simulink model "npc_diag"  (R2023b)
settings: Solver=FixedStepDiscrete  StartTime=0  StopTime=4  FixedStep=1e-06  RelTol=1e-3
libraries: spsThreePhaseSeriesRLCBranchLib x3, spsDCVoltageSourceLib x2, spsVoltageMeasurementLib x2, spsGroundLib x1, spsThreeLevelBridgeLib x1, spsPWMGenerator3LevelLib x1, spsThreePhaseVIMeasurementLib x1, spspowerguiLib x1
settings Model: Creator=ASUS  LastModifiedBy=ASUS
settings DataIOCC: SaveOutput=off  SaveTime=off

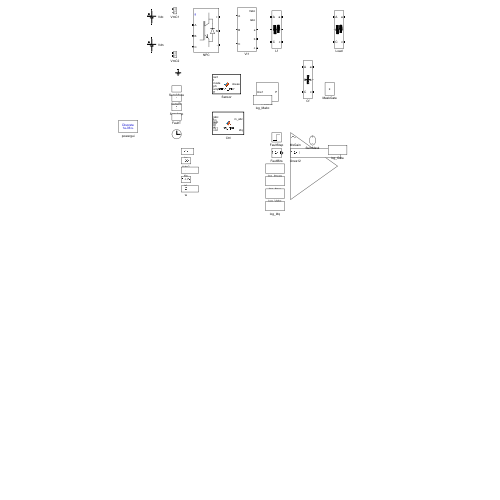
[thumbnail: Simulink's stored preview of the top-level diagram]
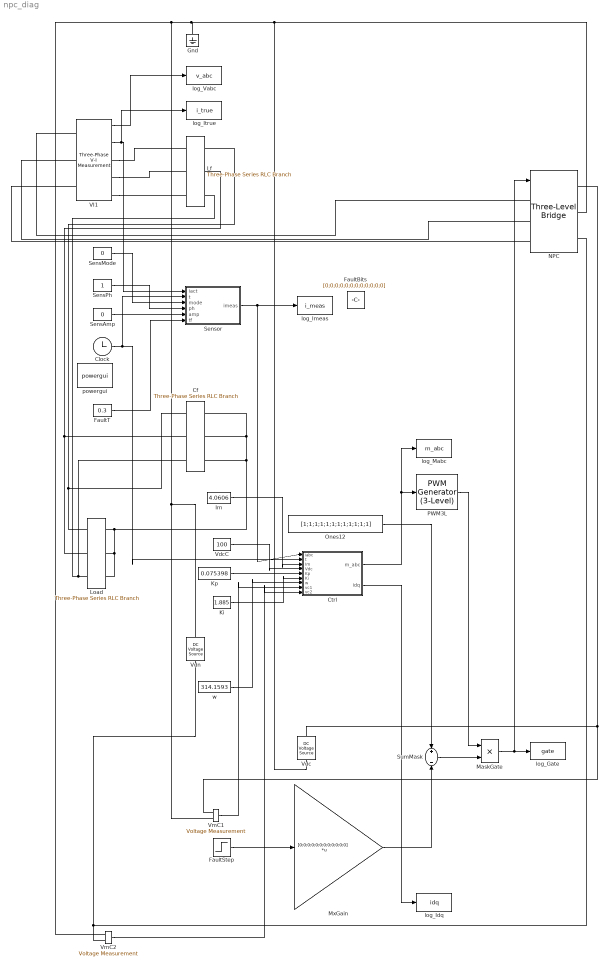
== system npc_diag ==
  Cf : spsThreePhaseSeriesRLCBranchLib/Three-Phase Series RLC Branch  LConnTagsString=A|B|C  RConnTagsString=A|B|C  BranchType=C  Resistance=1  Inductance=1e-3  Capacitance=5e-05  Measurements=None
  Clock : Clock
  Ctrl : MATLAB Function  TreatAsAtomicUnit=on
  FaultBits : Constant  Value=[0;0;0;0;0;0;0;0;0;0;0;0]
  FaultStep : Step  Time=0.3  SampleTime=0
  FaultT : Constant  Value=0.3
  Gnd : spsGroundLib/Ground  LConnTagsString=a
  Im : Constant  Value=4.0606
  Ki : Constant  Value=1.885
  Kp : Constant  Value=0.075398
  Lf : spsThreePhaseSeriesRLCBranchLib/Three-Phase Series RLC Branch  LConnTagsString=A|B|C  RConnTagsString=A|B|C  BranchType=RL  Resistance=0.05  Inductance=0.002  Capacitance=1e-6  Measurements=None
  Load : spsThreePhaseSeriesRLCBranchLib/Three-Phase Series RLC Branch  LConnTagsString=A|B|C  RConnTagsString=A|B|C  BranchType=RL  Resistance=10  Inductance=0  Capacitance=1e-6  Measurements=None
  MaskGate : Product
  MxGain : Gain  Gain=[0;0;0;0;0;0;0;0;0;0;0;0]  Multiplication=Matrix(K*u)
  NPC : spsThreeLevelBridgeLib/Three-Level Bridge  Arms=3  SnubberResistance=100000  SbubberCapacitance=inf  Device=IGBT / Diodes  Ron=0.001  ForwardVoltages=[0 0]  Measurements=None
  Ones12 : Constant  Value=[1;1;1;1;1;1;1;1;1;1;1;1]
  PWM3L : spsPWMGenerator3LevelLib/PWM Generator (3-Level)  ModulatorType=Three-phase bridge (12 pulses)  ModulatorMode=Unsynchronized  nF=200  Fc=10000  ModulatingSignals=off  m=0.8  Freq=50  Phase=0  Ts=0
  SensAmp : Constant  Value=0
  SensMode : Constant  Value=0
  SensPh : Constant
  Sensor : MATLAB Function  TreatAsAtomicUnit=on
  SumMask : Sum  Inputs=+-
  VI1 : spsThreePhaseVIMeasurementLib/Three-Phase V-I Measurement  VoltageMeasurement=phase-to-ground  SetLabelV=off  LabelV=Vabc  Vpu=off  VpuLL=off  CurrentMeasurement=yes  SetLabelI=off  LabelI=Iabc  Ipu=off  Pbase=100e6  Vbase=500e3  OutputType=Complex  PhasorSimulation=off  PSBequivalent=0
  Vdc : spsDCVoltageSourceLib/DC Voltage Source  Amplitude=50  Measurements=None
  VdcC : Constant  Value=100
  Vdn : spsDCVoltageSourceLib/DC Voltage Source  Amplitude=50  Measurements=None
  VmC1 : spsVoltageMeasurementLib/Voltage Measurement  PhasorSimulation=off  OutputType=Complex  PSBequivalent=0
  VmC2 : spsVoltageMeasurementLib/Voltage Measurement  PhasorSimulation=off  OutputType=Complex  PSBequivalent=0
  log_Gate : ToWorkspace  VariableName=gate  SaveFormat=Timeseries  SampleTime=5e-05
  log_Idq : ToWorkspace  VariableName=idq  SaveFormat=Timeseries  SampleTime=5e-05
  log_Imeas : ToWorkspace  VariableName=i_meas  SaveFormat=Timeseries  SampleTime=5e-05
  log_Itrue : ToWorkspace  VariableName=i_true  SaveFormat=Timeseries  SampleTime=5e-05
  log_Mabc : ToWorkspace  VariableName=m_abc  SaveFormat=Timeseries  SampleTime=5e-05
  log_Vabc : ToWorkspace  VariableName=v_abc  SaveFormat=Timeseries  SampleTime=5e-05
  powergui : spspowerguiLib/powergui  Priority=1  SimulationMode=Discrete  SampleTime=1e-06  frequency=60  Iterations=50  frequencyindice=0  Pbase=100e6  ErrMax=1e-4  UnitsV=kV  UnitsW=MW  buscounter=0  FunctionMessages=off  echomessages=off  EnableUseOfTLC=off  CurrentSourceSwitches=off  DisableSnubberDevices=off  DisableRonSwitches=off  DisableVfSwitches=off  DisplayEquations=off  AutomaticDiscreteSolvers=off  SolverType=Tustin/Backward Euler (TBE)  Interpol=off  ExternalGateDelay=off  methode=off  Ts=100  x0status=blocks  SPID=on  SwTol=0  HookPort=off  NonlinearTolerance=1e-4  nMaxIteration=100  ContinueOnMaxIteration=off  RestoreLinks=warning  ResistiveCurrentMeasurement=off  Frange=[0:2:500]  Ylog=off  Xlog=on  ShowGrid=off  save=off  variable=ZData  structure=0  ZoomFFT=off  StartTime=0.0  cycles=1  DisplayStyle=1  fundamental=60  FreqAxis=off  MaxFrequency=1000  frequencyindicesteady=1  RmsSteady=1  display=off
  w : Constant  Value=314.1593
  wires:
  SumMask/1 -> MaskGate/2
  FaultStep/1 -> MxGain/1
  Sensor/1(imeas) -> Ctrl/1(iabc), log_Imeas/1
  VI1/1 -> log_Vabc/1
  VI1/2 -> Sensor/1(iact), log_Itrue/1
  Kp/1 -> Ctrl/5(Kp)
  SensAmp/1 -> Sensor/5(amp)
  Im/1 -> Ctrl/3(Im)
  FaultT/1 -> Sensor/6(tf)
  SensMode/1 -> Sensor/3(mode)
  SensPh/1 -> Sensor/4(ph)
  Clock/1 -> Ctrl/2(t), Sensor/2(t)
  VmC2/1 -> Ctrl/9(vc2)
  VdcC/1 -> Ctrl/4(Vdc)
  Ki/1 -> Ctrl/6(Ki)
  w/1 -> Ctrl/7(w)
  VmC1/1 -> Ctrl/8(vc1)
  Ones12/1 -> SumMask/1
  Ctrl/1(m_abc) -> PWM3L/1, log_Mabc/1
  Ctrl/2(idq) -> log_Idq/1
  MxGain/1 -> SumMask/2
  PWM3L/1 -> MaskGate/1
  MaskGate/1 -> NPC/1, log_Gate/1
  connections:
  Load/LConn1 -- Lf/RConn1 -- Cf/LConn1
  Load/LConn2 -- Lf/RConn2 -- Cf/LConn2
  Load/LConn3 -- Lf/RConn3 -- Cf/LConn3
  VmC2/LConn1 -- Vdn/RConn1 -- VmC1/LConn2 -- NPC/RConn2 -- Vdc/LConn1 -- Gnd/LConn1
  VmC2/LConn2 -- Vdn/LConn1 -- NPC/RConn3
  NPC/LConn2 -- VI1/LConn2
  VI1/RConn1 -- Lf/LConn1
  VI1/RConn2 -- Lf/LConn2
  VI1/RConn3 -- Lf/LConn3
  NPC/LConn3 -- VI1/LConn3
  VmC1/LConn1 -- NPC/RConn1 -- Vdc/RConn1
  Load/RConn1 -- Load/RConn3 -- Load/RConn2 -- Cf/RConn1 -- Cf/RConn2 -- Cf/RConn3
  NPC/LConn1 -- VI1/LConn1

== matlab function npc_diag/Ctrl ==
  data: iabc input; m_abc output; t input; Im input; Vdc input; Kp input; Ki input; w input; vc1 input; vc2 input; idq output
function [m_abc, idq] = ctrl_npc(iabc, t, Im, Vdc, Kp, Ki, w, vc1, vc2)
%CTRL_NPC  20 kHz sampled dq PI controller, called by a 1 us plant solver.
% Version: sampled-zoh-v4. All outputs are held between integer 50 us ticks.
% Integrate the previous sampled error over its hold time. Saturated intervals
% freeze the integral but ALWAYS advance the clock. No fictitious startup dt.
%#codegen
Ts = 50e-6;
Lf = 2e-3;
K_NP = 0.004;
M_NP_MAX = 0.12;
persistent xi last_tick last_update last_call old_error allow_integral m_hold dq_hold
if isempty(xi)
    xi = zeros(2,1);
    last_tick = -1;
    last_update = t;
    last_call = t;
    old_error = zeros(2,1);
    allow_integral = false;
    m_hold = zeros(3,1);
    dq_hold = zeros(2,1);
end
if t < last_call - 1e-12
    xi = zeros(2,1);
    last_tick = -1;
    last_update = t;
    old_error = zeros(2,1);
    allow_integral = false;
    m_hold = zeros(3,1);
    dq_hold = zeros(2,1);
end
last_call = t;
% Tiny tolerance only removes floating point boundary error (5 ps).
tick = floor(t / Ts + 1e-7);
if tick == last_tick
    m_abc = m_hold;
    idq = dq_hold;
    return
end
dt = t - last_update;
if last_tick >= 0 && allow_integral
    xi = xi + old_error * dt;
end
last_update = t;                 % advance even while saturated
last_tick = tick;
th = w*t;
c = [cos(th); cos(th-2*pi/3); cos(th+2*pi/3)];
s = [sin(th); sin(th-2*pi/3); sin(th+2*pi/3)];
id = (2/3)*(c'*iabc);
iq = -(2/3)*(s'*iabc);
err = [Im-id; -iq];
md = Kp*err(1) + Ki*xi(1) + (2*w*Lf/Vdc)*iq;
mq = Kp*err(2) + Ki*xi(2) - (2*w*Lf/Vdc)*id;
cm = max(min(-K_NP*(vc1-vc2), M_NP_MAX), -M_NP_MAX);
raw = md*c - mq*s + cm;
allow_integral = abs(md) <= 1 && abs(mq) <= 1 && all(abs(raw) <= 1);
old_error = err;
md = max(min(md,1),-1);
mq = max(min(mq,1),-1);
m_hold = max(min(md*c-mq*s+cm,1),-1);
dq_hold = [id;iq];
m_abc = m_hold;
idq = dq_hold;
end

== matlab function npc_diag/Sensor ==
  data: iact input; imeas output; t input; mode input; ph input; amp input; tf input
function imeas = sensor_fault(iact, t, mode, ph, amp, tf)
%SENSOR_FAULT  三相电流传感器故障模型
%
%   说明：传感器是代数模型，不涉及积分，因此不需要时间门控（块按 1 µs 执行不影响
%   正确性，只是把同一采样值重复算了几十次）。保留最简单的单出口结构，便于代码生成。
%
%   输入：iact(3x1) 真实电流, t 时间, mode 0=N/1=DF/2=SF/3=OF,
%         ph 故障相, amp OF 偏置幅度, tf 故障注入时刻
%   输出：imeas(3x1) 传感器输出（送控制器 + 作为诊断输入记录）

%#codegen
persistent held
if isempty(held)
    held = zeros(3,1);
end

imeas = iact;
if t < tf
    held = iact;          % 故障前持续跟踪真实值
else
    for k = 1:3
        if k == ph
            if mode == 1
                imeas(k) = 0;              % 断线
            elseif mode == 2
                imeas(k) = held(k);        % 卡死
            elseif mode == 3
                imeas(k) = iact(k) + amp;  % 偏置
            end
        end
    end
end
end
